simulink model "MSD_with_force"  (R2025b)
settings: Solver=ode8  StartTime=0.0  StopTime=10  FixedStep=0.01  RelTol=1e-3
InitFcn:
  | m=10;
  | k=100;
  | d=10;
settings Model: Creator=MehrSystem  LastModifiedBy=MehrSystem

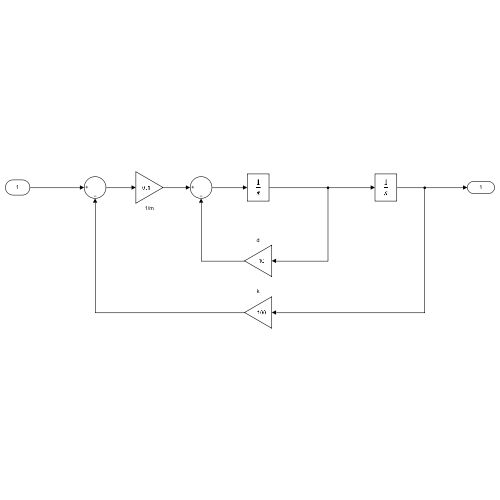
[thumbnail: Simulink's stored preview of the top-level diagram]
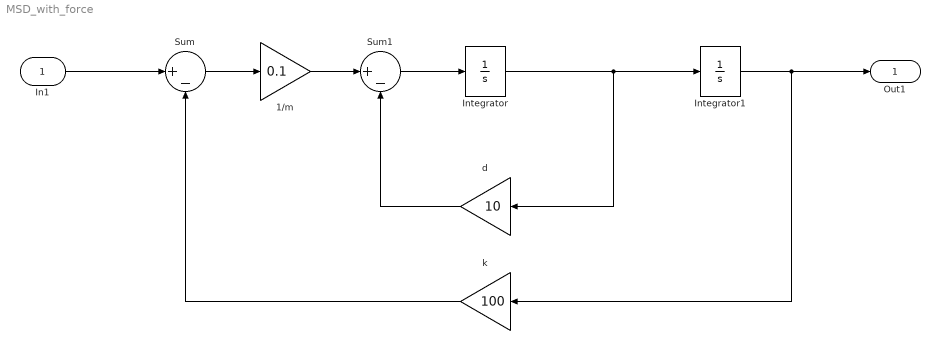
== system MSD_with_force ==
  In1 : Inport
  1/m : Gain  Gain=0.1
  Integrator : Integrator
  Integrator1 : Integrator
  Sum : Sum  Inputs=|+-
  Sum1 : Sum  Inputs=|+-
  d : Gain  Gain=10
  k : Gain  Gain=100
  Out1 : Outport
  wires:
  In1/1 -> Sum/1
  k/1 -> Sum/2
  Sum/1 -> 1/m/1
  1/m/1 -> Sum1/1
  Sum1/1 -> Integrator/1
  Integrator/1 -> Integrator1/1, d/1
  d/1 -> Sum1/2
  Integrator1/1 -> Out1/1, k/1
